simulink model "dofstuff"  (R2026b)
settings: Solver=ode4  StopTime=60  FixedStep=0.02
undefined symbols (not defined in the file): dragCoeffVec, g, Kdtheta, Kdz, Kitheta, Kiz, Kptheta, Kpz, m, rho
libraries: aerolibanimutils x1, uavutilslib x1
settings Model: SimulationMode=accelerator  Creator=YoYo  LastModifiedBy=YoYo
settings SolverCC: MinimalZcImpactIntegration=on
settings DataIOCC: DSMLogging=off  ReturnWorkspaceOutputs=off  SaveOutput=off  SaveTime=off  SignalLogging=off
settings DebuggingCC: MultiTaskDSMMsg=none  ReadBeforeWriteMsg=DisableAll  WriteAfterReadMsg=DisableAll  WriteAfterWriteMsg=DisableAll
settings SFSimCC: SFSimEcho=off

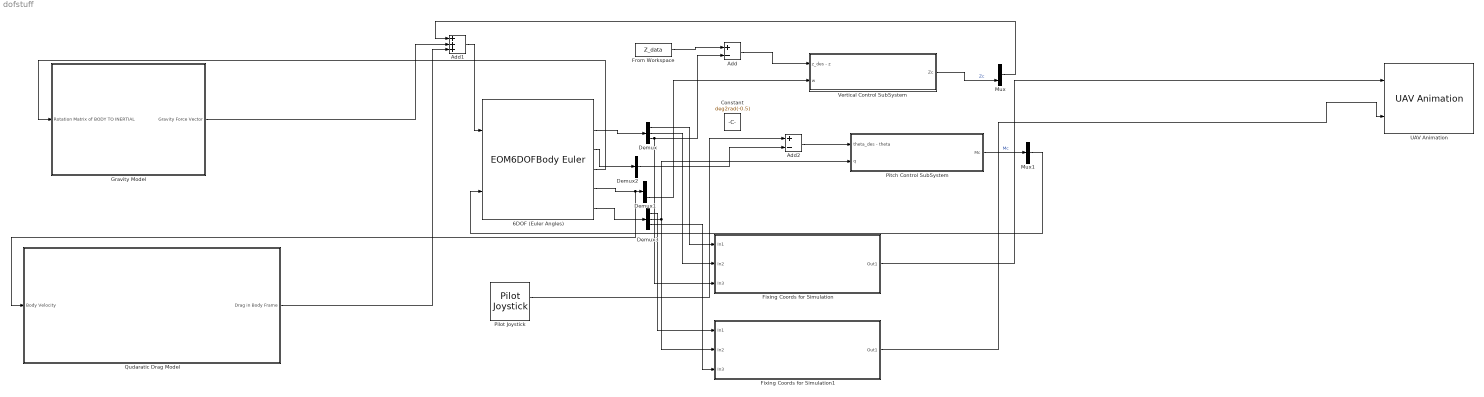
== system dofstuff ==
  6DOF (Euler Angles) : EOM6DOFBodyEuler  mass_0=5.6
  Add : Sum  Inputs=+-
  Add1 : Sum  Inputs=+++
  Add2 : Sum  Inputs=+-
  Constant : Constant  Value=deg2rad(-0.5)
  Demux{,1..3} (4 alike) : Demux  Outputs=3
  Fixing Coords for Simulation : Subsystem  Priority=-1
  Fixing Coords for Simulation1 : Subsystem  Priority=-1
  From Workspace : FromWorkspace  VariableName=Z_data
  Gravity Model : Subsystem
  Mux : Mux  Inputs=3
  Mux1 : Mux  Inputs=3
  Pilot Joystick : aerolibanimutils/Pilot Joystick  JoystickID=Joystick1  OutputConfiguration=FourAxis  SampleTime=0.02  action=Error
  Pitch Control SubSystem : Subsystem
  Qudaratic Drag Model : Subsystem
  UAV Animation : uavutilslib/UAV Animation  NumUAV=1  DynamicUAVConfig=off  UAVType=Multirotor  UAVSize=1  UAVColor=[1 0 0]  UAVTrajectoryAlpha=1  AlwaysShowAnimation=on  AxisLimits=[-Inf Inf;-Inf Inf;-Inf Inf]  TrajectoryBufferSize=500  InertialZDirection=Up  RotationFormat=Euler ZYX  DrawMarkers=off  SampleTime=0.02
  Vertical Control SubSystem : Subsystem
  wires:
  6DOF (Euler Angles)/2 -> Demux/1
  From Workspace/1 -> Add/1
  Demux/3 -> Fixing Coords for Simulation/3(In3), Add/2
  Add/1 -> Vertical Control SubSystem/1(z_des - z)
  6DOF (Euler Angles)/5 -> Qudaratic Drag Model/1(Body Velocity), Demux1/1
  Demux1/3 -> Vertical Control SubSystem/2(w)
  Vertical Control SubSystem/1(Zc) -> Mux/3  "Zc"
  Mux/1 -> Add1/1
  Add1/1 -> 6DOF (Euler Angles)/1
  6DOF (Euler Angles)/4 -> Gravity Model/1(Rotation Matrix of BODY TO INERTIAL)
  Gravity Model/1(Gravity Force Vector) -> Add1/2
  Qudaratic Drag Model/1(Drag in Body Frame) -> Add1/3
  6DOF (Euler Angles)/3 -> Demux2/1
  Demux2/2 -> Add2/2
  Add2/1 -> Pitch Control SubSystem/1(theta_des - theta)
  6DOF (Euler Angles)/6 -> Demux3/1
  Demux3/2 -> Fixing Coords for Simulation1/2(In2), Pitch Control SubSystem/2(q)
  Pitch Control SubSystem/1(Mc) -> Mux1/2  "Mc"
  Mux1/1 -> 6DOF (Euler Angles)/2
  Demux/1 -> Fixing Coords for Simulation/1(In1)
  Demux/2 -> Fixing Coords for Simulation/2(In2)
  Demux3/1 -> Fixing Coords for Simulation1/1(In1)
  Demux3/3 -> Fixing Coords for Simulation1/3(In3)
  Fixing Coords for Simulation/1(Out1) -> UAV Animation/1
  Fixing Coords for Simulation1/1(Out1) -> UAV Animation/2
  Pilot Joystick/2 -> Add2/1

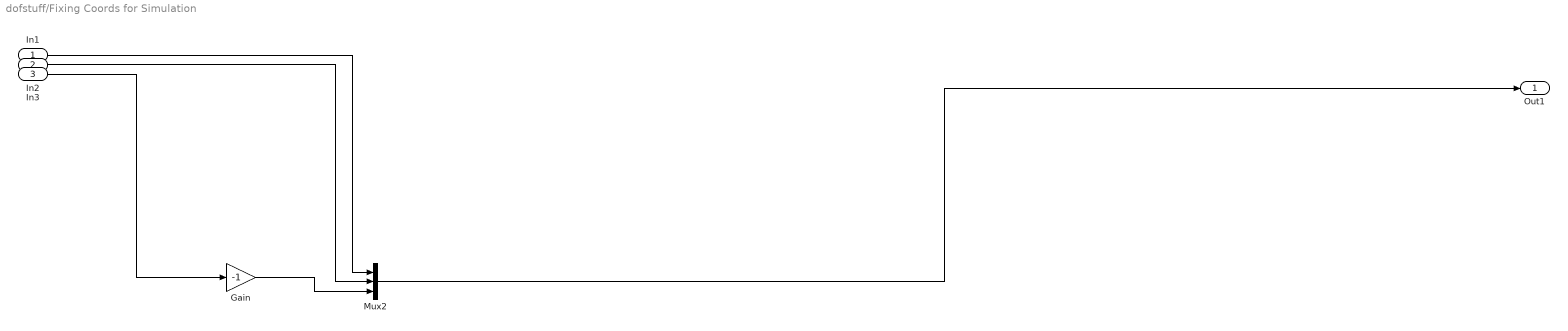
== system dofstuff/Fixing Coords for Simulation ==
  In1 : Inport
  In2 : Inport  Port=2
  In3 : Inport  Port=3
  Gain : Gain  Gain=-1
  Mux2 : Mux  Inputs=3
  Out1 : Outport
  wires:
  Mux2/1 -> Out1/1
  In2/1 -> Mux2/2
  Gain/1 -> Mux2/3
  In1/1 -> Mux2/1
  In3/1 -> Gain/1

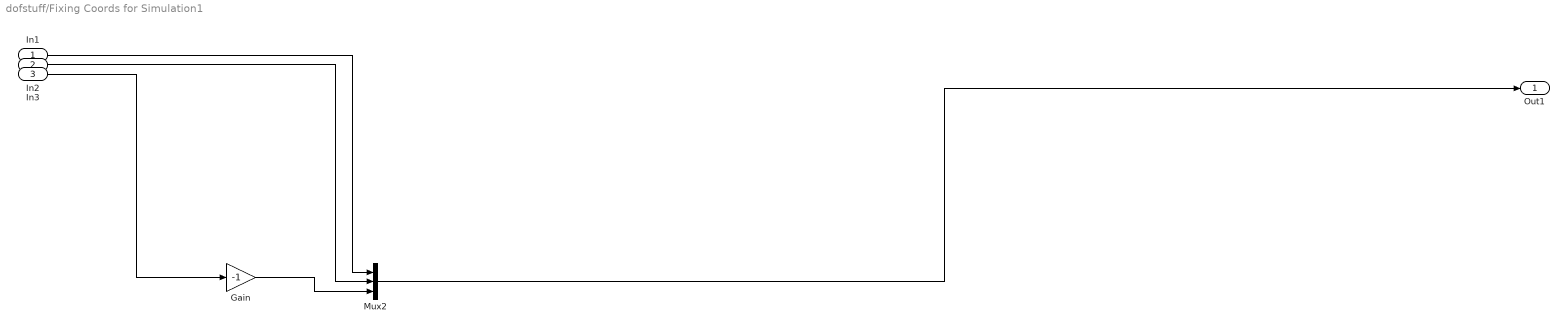
== system dofstuff/Fixing Coords for Simulation1 ==
  In1 : Inport
  In2 : Inport  Port=2
  In3 : Inport  Port=3
  Gain : Gain  Gain=-1
  Mux2 : Mux  Inputs=3
  Out1 : Outport
  wires:
  Mux2/1 -> Out1/1
  In2/1 -> Mux2/2
  Gain/1 -> Mux2/3
  In1/1 -> Mux2/1
  In3/1 -> Gain/1

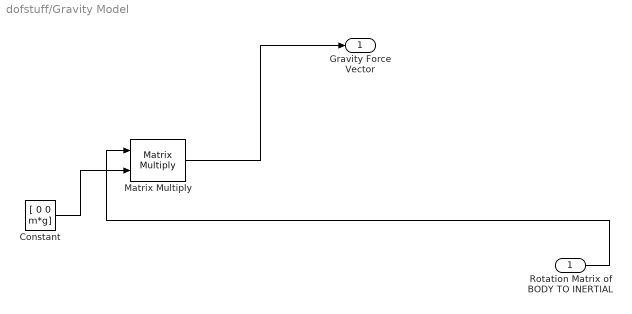
== system dofstuff/Gravity Model ==
  Rotation Matrix of BODY TO INERTIAL : Inport
  Constant : Constant  Value=[ 0 0 m*g]
  Matrix Multiply : Product  Multiplication=Matrix(*)
  Gravity Force Vector : Outport
  wires:
  Constant/1 -> Matrix Multiply/2
  Rotation Matrix of BODY TO INERTIAL/1 -> Matrix Multiply/1
  Matrix Multiply/1 -> Gravity Force Vector/1

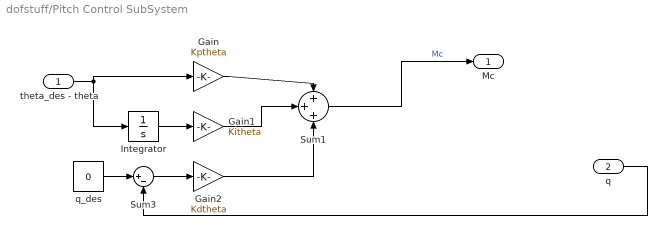
== system dofstuff/Pitch Control SubSystem ==
  theta_des - theta : Inport
  q : Inport  Port=2
  Gain : Gain  Gain=Kptheta
  Gain1 : Gain  Gain=Kitheta
  Gain2 : Gain  Gain=Kdtheta
  Integrator : Integrator  LimitOutput=on  UpperSaturationLimit=500  LowerSaturationLimit=-500
  Sum1 : Sum  Inputs=+++
  Sum3 : Sum  Inputs=|+-
  q_des : Constant  Value=0
  Mc : Outport
  wires:
  Sum1/1 -> Mc/1  "Mc"
  theta_des - theta/1 -> Integrator/1, Gain/1
  q/1 -> Sum3/2
  Gain/1 -> Sum1/1
  Sum3/1 -> Gain2/1
  Integrator/1 -> Gain1/1
  q_des/1 -> Sum3/1
  Gain1/1 -> Sum1/2
  Gain2/1 -> Sum1/3

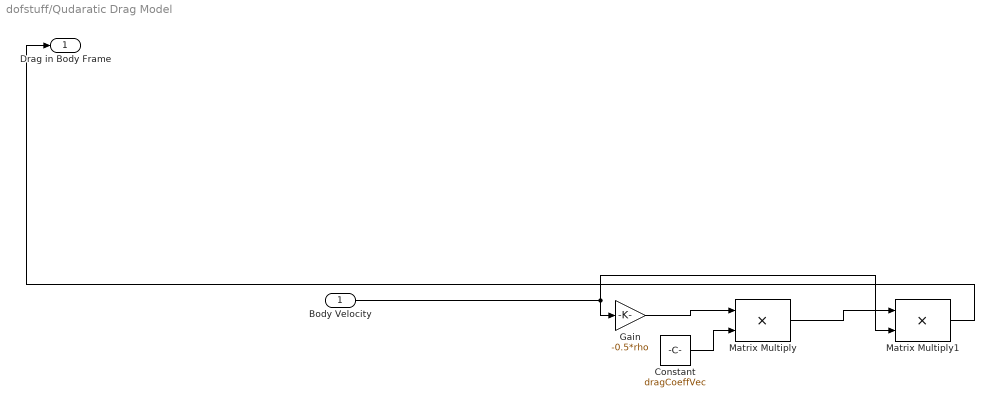
== system dofstuff/Qudaratic Drag Model ==
  Body Velocity : Inport
  Constant : Constant  Value=dragCoeffVec
  Gain : Gain  Gain=-0.5*rho
  Matrix Multiply : Product
  Matrix Multiply1 : Product
  Drag in Body Frame : Outport
  wires:
  Matrix Multiply/1 -> Matrix Multiply1/1
  Gain/1 -> Matrix Multiply/1
  Body Velocity/1 -> Gain/1, Matrix Multiply1/2
  Constant/1 -> Matrix Multiply/2
  Matrix Multiply1/1 -> Drag in Body Frame/1

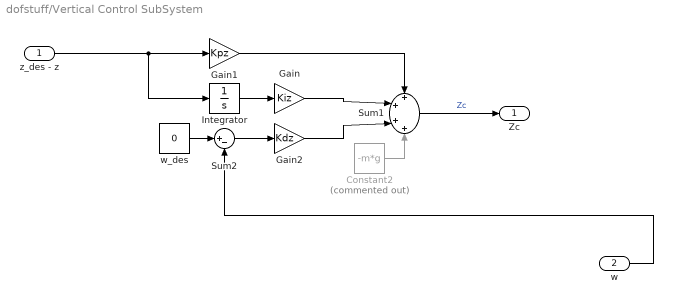
== system dofstuff/Vertical Control SubSystem ==
  z_des - z : Inport
  w : Inport  Port=2
  Constant2 : Constant  Commented=on  Value=-m*g
  Gain : Gain  Gain=Kiz
  Gain1 : Gain  Gain=Kpz
  Gain2 : Gain  Gain=Kdz
  Integrator : Integrator  LimitOutput=on  UpperSaturationLimit=500  LowerSaturationLimit=-500
  Sum1 : Sum  Inputs=++++
  Sum2 : Sum  Inputs=|+-
  w_des : Constant  Value=0
  Zc : Outport
  wires:
  w/1 -> Sum2/2
  Constant2/1 -> Sum1/4
  Gain1/1 -> Sum1/1
  Sum1/1 -> Zc/1  "Zc"
  w_des/1 -> Sum2/1
  Integrator/1 -> Gain/1
  z_des - z/1 -> Integrator/1, Gain1/1
  Sum2/1 -> Gain2/1
  Gain2/1 -> Sum1/3
  Gain/1 -> Sum1/2
